simulink model "DCMotor_M2_PISim"  (R2026b)
settings: Solver=FixedStepDiscrete  StopTime=Ref_StopTime  FixedStep=Ts
PreLoadFcn:
  | DCMotorParams;
InitFcn:
  | DCMotorParams;
values from neighbouring files (symbols this model uses):
  Duty_Coulomb = 1.024    [DCMotorParams.m]
  Enc_RPMGain = Enc_Dir*Enc_Kcal*60/(Ts*Enc_CountsPerRev)    (= 23.5340909091)    [DCMotorParams.m]
  RPM_LPF_Den = [1, RPM_LPF_a - 1]    [DCMotorParams.m]
  RPM_LPF_Num = RPM_LPF_a    (= 0.2)    [DCMotorParams.m]
  Sim_DutyBreakaway = 14.0    (= 14)    [DCMotorParams.m]
  Sim_FrictionEnable = 1    [DCMotorParams.m]
  Sim_StickRPM = 5    [DCMotorParams.m]
  Ts = 0.01    [DCMotorParams.m]
undefined symbols (not defined in the file or in its folder): DiscIntNeverNeededParam, Plant_Den, Plant_Num
libraries: simulink x1
settings Model: Creator=bence  LastModifiedBy=bence

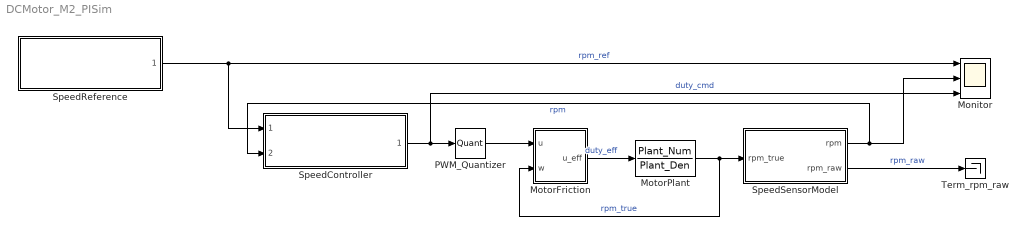
== system DCMotor_M2_PISim ==
  Monitor : Scope  NumInputPorts=3
  MotorFriction : MATLAB Function  TreatAsAtomicUnit=on
  MotorPlant : DiscreteTransferFcn  Numerator=Plant_Num  Denominator=Plant_Den  SampleTime=Ts
  PWM_Quantizer : Quantizer  QuantizationInterval=Duty_Quant
  SpeedController : Subsystem  ReferencedSubsystem=SpeedController
  SpeedReference : Subsystem  ReferencedSubsystem=SpeedReference
  SpeedSensorModel : Subsystem
  Term_rpm_raw : Terminator
  wires:
  SpeedSensorModel/2(rpm_raw) -> Term_rpm_raw/1  "rpm_raw"
  SpeedSensorModel/1(rpm) -> Monitor/2, SpeedController/2  "rpm"
  SpeedReference/1 -> SpeedController/1, Monitor/1  "rpm_ref"
  MotorFriction/1(u_eff) -> MotorPlant/1  "duty_eff"
  PWM_Quantizer/1 -> MotorFriction/1(u)
  SpeedController/1 -> Monitor/3, PWM_Quantizer/1  "duty_cmd"
  MotorPlant/1 -> MotorFriction/2(w), SpeedSensorModel/1(rpm_true)  "rpm_true"

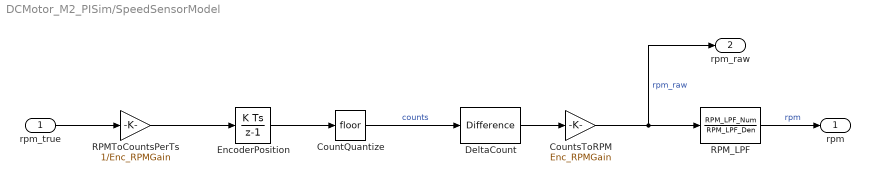
== system DCMotor_M2_PISim/SpeedSensorModel ==
  rpm_true : Inport
  CountQuantize : Rounding
  CountsToRPM : Gain  Gain=Enc_RPMGain
  DeltaCount : simulink/Discrete/Difference  ICPrevInput=0.0  OutMin=[]  OutMax=[]  OutDataType=fixdt(1, 16)  OutScaling=2^-10  DoSatur=off
  EncoderPosition : DiscreteIntegrator  gainval=1/Ts  SampleTime=Ts  ICPrevOutput=DiscIntNeverNeededParam  ICPrevScaledInput=DiscIntNeverNeededParam
  RPMToCountsPerTs : Gain  Gain=1/Enc_RPMGain
  RPM_LPF : DiscreteTransferFcn  Numerator=RPM_LPF_Num  Denominator=RPM_LPF_Den  SampleTime=Ts
  rpm : Outport
  rpm_raw : Outport  Port=2
  wires:
  RPM_LPF/1 -> rpm/1  "rpm"
  CountsToRPM/1 -> RPM_LPF/1, rpm_raw/1  "rpm_raw"
  DeltaCount/1 -> CountsToRPM/1
  CountQuantize/1 -> DeltaCount/1  "counts"
  EncoderPosition/1 -> CountQuantize/1
  RPMToCountsPerTs/1 -> EncoderPosition/1
  rpm_true/1 -> RPMToCountsPerTs/1

== matlab function DCMotor_M2_PISim/MotorFriction ==
  data: u input; u_eff output; w input; Sim_FrictionEnable parameter; Duty_Coulomb parameter; Sim_DutyBreakaway parameter; Sim_StickRPM parameter
function u_eff = MotorFriction(u, w, Sim_FrictionEnable, Duty_Coulomb, Sim_DutyBreakaway, Sim_StickRPM)
%MOTORFRICTION Static + Coulomb friction acting on the duty command (simulation only).
%   Standstill (|w| < Sim_StickRPM): motor stays stuck until |u| > Sim_DutyBreakaway.
%   Moving: Coulomb friction removes Duty_Coulomb in the direction of motion.
if Sim_FrictionEnable == 0
    u_eff = u;
elseif abs(w) < Sim_StickRPM
    if abs(u) <= Sim_DutyBreakaway
        u_eff = 0;
    else
        u_eff = u - sign(u)*Duty_Coulomb;
    end
else
    u_eff = u - sign(w)*Duty_Coulomb;
end
end
